simulink model "Exp4_Home_ELD_Hopfield_vs_Lambda"  (R2025b)
settings: Solver=FixedStepDiscrete  StartTime=0  StopTime=23  FixedStep=1  RelTol=1e-3
libraries: simulink x3
settings Model: Creator=mithu  LastModifiedBy=mithu

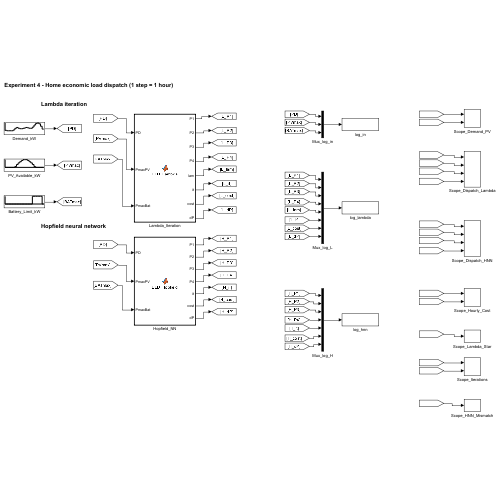
[thumbnail: Simulink's stored preview of the top-level diagram]
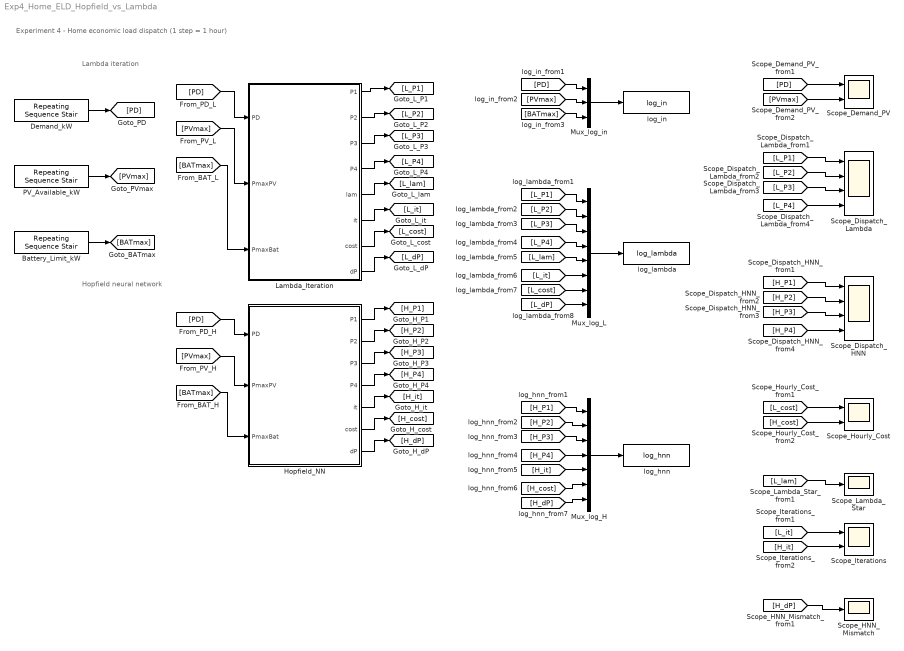
== system Exp4_Home_ELD_Hopfield_vs_Lambda ==
  note: Experiment 4 - Home economic load dispatch (1 step = 1 hour)
  note: Lambda iteration
  note: Hopfield neural network
  Battery_Limit_kW : simulink/Sources/Repeating Sequence Stair  OutValues=Exp4_battlim  tsamp=1  OutMin=[]  OutMax=[]  OutDataTypeStr=double  OutputDataTypeScalingMode=double  OutDataType=fixdt(0,8)  ConRadixGroup=Best Precision: Vector-wise  OutScaling=2^-12
  Demand_kW : simulink/Sources/Repeating Sequence Stair  OutValues=Exp4_load  tsamp=1  OutMin=[]  OutMax=[]  OutDataTypeStr=double  OutputDataTypeScalingMode=double  OutDataType=fixdt(0,8)  ConRadixGroup=Best Precision: Vector-wise  OutScaling=2^-12
  Hopfield_NN : MATLAB Function  TreatAsAtomicUnit=on
  Lambda_Iteration : MATLAB Function  TreatAsAtomicUnit=on
  Mux_log_H : Mux  Inputs=7
  Mux_log_L : Mux  Inputs=8
  Mux_log_in : Mux  Inputs=3
  PV_Available_kW : simulink/Sources/Repeating Sequence Stair  OutValues=Exp4_pv  tsamp=1  OutMin=[]  OutMax=[]  OutDataTypeStr=double  OutputDataTypeScalingMode=double  OutDataType=fixdt(0,8)  ConRadixGroup=Best Precision: Vector-wise  OutScaling=2^-12
  Scope_Demand_PV : Scope  NumInputPorts=2
  Scope_Dispatch_HNN : Scope  NumInputPorts=4
  Scope_Dispatch_Lambda : Scope  NumInputPorts=4
  Scope_HNN_Mismatch : Scope
  Scope_Hourly_Cost : Scope  NumInputPorts=2
  Scope_Iterations : Scope  NumInputPorts=2
  Scope_Lambda_Star : Scope
  log_hnn : ToWorkspace  VariableName=log_hnn  SaveFormat=Timeseries  SampleTime=1
  log_in : ToWorkspace  VariableName=log_in  SaveFormat=Timeseries  SampleTime=1
  log_lambda : ToWorkspace  VariableName=log_lambda  SaveFormat=Timeseries  SampleTime=1
  wires:
  Demand_kW/1 -> [PD]
  PV_Available_kW/1 -> [PVmax]
  Battery_Limit_kW/1 -> [BATmax]
  [PD] -> Lambda_Iteration/1(PD)
  [PVmax] -> Lambda_Iteration/2(PmaxPV)
  [BATmax] -> Lambda_Iteration/3(PmaxBat)
  [PD] -> Hopfield_NN/1(PD)
  [PVmax] -> Hopfield_NN/2(PmaxPV)
  [BATmax] -> Hopfield_NN/3(PmaxBat)
  Lambda_Iteration/1(P1) -> [L_P1]
  Lambda_Iteration/2(P2) -> [L_P2]
  Lambda_Iteration/3(P3) -> [L_P3]
  Lambda_Iteration/4(P4) -> [L_P4]
  Lambda_Iteration/5(lam) -> [L_lam]
  Lambda_Iteration/6(it) -> [L_it]
  Lambda_Iteration/7(cost) -> [L_cost]
  Lambda_Iteration/8(dP) -> [L_dP]
  Hopfield_NN/1(P1) -> [H_P1]
  Hopfield_NN/2(P2) -> [H_P2]
  Hopfield_NN/3(P3) -> [H_P3]
  Hopfield_NN/4(P4) -> [H_P4]
  Hopfield_NN/5(it) -> [H_it]
  Hopfield_NN/6(cost) -> [H_cost]
  Hopfield_NN/7(dP) -> [H_dP]
  [PD] -> Mux_log_in/1
  [PVmax] -> Mux_log_in/2
  [BATmax] -> Mux_log_in/3
  Mux_log_in/1 -> log_in/1
  [L_P1] -> Mux_log_L/1
  [L_P2] -> Mux_log_L/2
  [L_P3] -> Mux_log_L/3
  [L_P4] -> Mux_log_L/4
  [L_lam] -> Mux_log_L/5
  [L_it] -> Mux_log_L/6
  [L_cost] -> Mux_log_L/7
  [L_dP] -> Mux_log_L/8
  Mux_log_L/1 -> log_lambda/1
  [H_P1] -> Mux_log_H/1
  [H_P2] -> Mux_log_H/2
  [H_P3] -> Mux_log_H/3
  [H_P4] -> Mux_log_H/4
  [H_it] -> Mux_log_H/5
  [H_cost] -> Mux_log_H/6
  [H_dP] -> Mux_log_H/7
  Mux_log_H/1 -> log_hnn/1
  [PD] -> Scope_Demand_PV/1
  [PVmax] -> Scope_Demand_PV/2
  [L_P1] -> Scope_Dispatch_Lambda/1
  [L_P2] -> Scope_Dispatch_Lambda/2
  [L_P3] -> Scope_Dispatch_Lambda/3
  [L_P4] -> Scope_Dispatch_Lambda/4
  [H_P1] -> Scope_Dispatch_HNN/1
  [H_P2] -> Scope_Dispatch_HNN/2
  [H_P3] -> Scope_Dispatch_HNN/3
  [H_P4] -> Scope_Dispatch_HNN/4
  [L_cost] -> Scope_Hourly_Cost/1
  [H_cost] -> Scope_Hourly_Cost/2
  [L_lam] -> Scope_Lambda_Star/1
  [L_it] -> Scope_Iterations/1
  [H_it] -> Scope_Iterations/2
  [H_dP] -> Scope_HNN_Mismatch/1

== matlab function Exp4_Home_ELD_Hopfield_vs_Lambda/Hopfield_NN ==
  data: PD input; P1 output; PmaxPV input; PmaxBat input; P2 output; P3 output; P4 output; it output; cost output; dP output
function [P1,P2,P3,P4,it,cost,dP] = ELD_Hopfield(PD,PmaxPV,PmaxBat)
% Hopfield neural-network economic dispatch for one hour
b = [0.5 3 6 25];  c = [0.02 0.4 0.3 1];  Pmin = [0 0 0 0];
Pmax = [PmaxPV PmaxBat 3 3];
A = 1;  B = 5e-4;  u0 = 1;  tol = 1e-7;  maxit = 100000;
rg  = max(Pmax-Pmin,1e-9);
eta = 0.9/(A*sum(rg)/(2*u0));
U = zeros(1,4);  V = Pmin + 0.5*rg;  q = 0;
for q = 1:maxit
    g  = -A*(PD-sum(V)) + (B/2)*(b + 2*c.*V);
    U  = U - eta*g;
    Vn = Pmin + 0.5*rg.*(1+tanh(U/u0));
    if max(abs(Vn-V)) < tol
        V = Vn;
        break
    end
    V = Vn;
end
P1 = V(1);  P2 = V(2);  P3 = V(3);  P4 = V(4);
it = q;
cost = sum(b.*V + c.*V.^2);
dP = PD - sum(V);
end

== matlab function Exp4_Home_ELD_Hopfield_vs_Lambda/Lambda_Iteration ==
  data: PD input; P1 output; PmaxPV input; PmaxBat input; P2 output; P3 output; P4 output; lam output; it output; cost output; dP output
function [P1,P2,P3,P4,lam,it,cost,dP] = ELD_Lambda(PD,PmaxPV,PmaxBat)
% Lambda-iteration economic dispatch for one hour
b = [0.5 3 6 25];  c = [0.02 0.4 0.3 1];  Pmin = [0 0 0 0];
Pmax = [PmaxPV PmaxBat 3 3];
tol = 1e-6;  maxit = 100;
lo = min(b + 2*c.*Pmin);  hi = max(b + 2*c.*Pmax);  L = (lo+hi)/2;
P = zeros(1,4);  k = 0;
for k = 1:maxit
    P = min(max((L-b)./(2*c),Pmin),Pmax);
    d = PD - sum(P);
    if abs(d) < tol
        break
    end
    if d > 0
        lo = L;
    else
        hi = L;
    end
    free = (P > Pmin+1e-12) & (P < Pmax-1e-12);
    if any(free)
        Ln = L + d/sum(1./(2*c(free)));
    else
        Ln = Inf;
    end
    if Ln > lo && Ln < hi
        L = Ln;
    else
        L = (lo+hi)/2;
    end
end
P1 = P(1);  P2 = P(2);  P3 = P(3);  P4 = P(4);
lam = L;  it = k;
cost = sum(b.*P + c.*P.^2);
dP = PD - sum(P);
end
